simulink model "omx_joint_state_monitor"  (R2026a)
settings: Solver=VariableStepAuto  StopTime=Inf
libraries: ros2lib x2
settings Model: Creator=parkjuwon  LastModifiedBy=parkjuwon

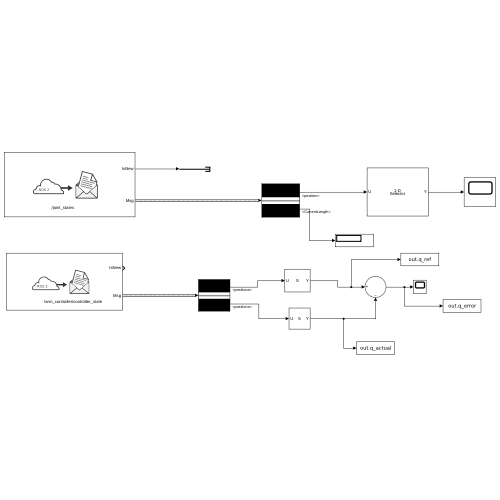
[thumbnail: Simulink's stored preview of the top-level diagram]
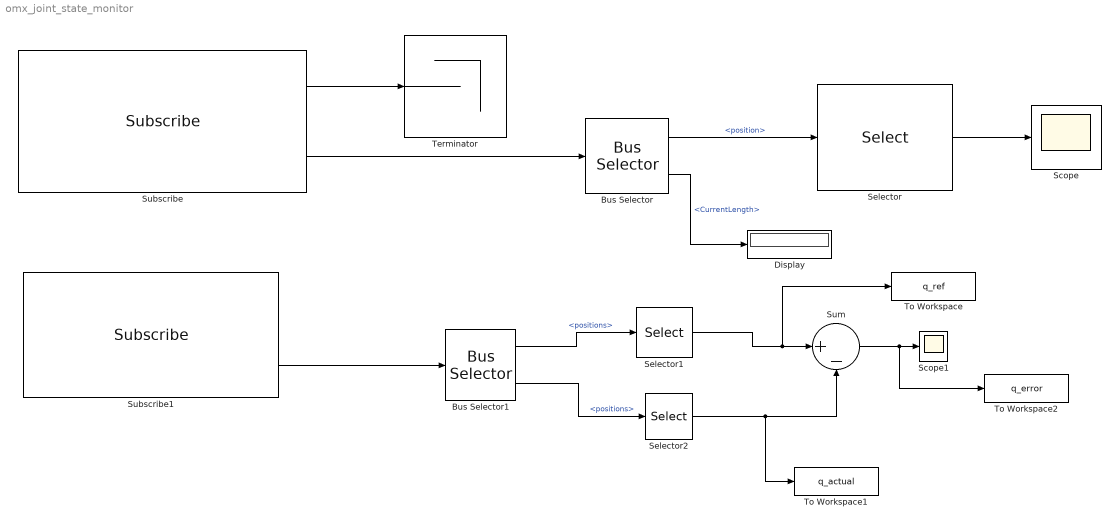
== system omx_joint_state_monitor ==
  Bus Selector : BusSelector  OutputSignals=position,position_SL_Info.CurrentLength
  Bus Selector1 : BusSelector  OutputSignals=reference.positions,feedback.positions
  Display : Display
  Scope : Scope
      settings: ActiveDisplayYMinimum=-1.1821267591514704  ActiveDisplayYMaximum=3.6890485001597582
  Scope1 : Scope
      settings: ActiveDisplayYMinimum=-6.9128041129529514  ActiveDisplayYMaximum=10.384679260876181
  Selector : Selector  IndexOptions=Index vector (dialog)  Indices=[3 4 5 6 7]  OutputSizes=1
  Selector1 : Selector  IndexOptions=Index vector (dialog)  Indices=[1 2 3 4 5]  OutputSizes=1
  Selector2 : Selector  IndexOptions=Index vector (dialog)  Indices=[1 2 3 4 5]  OutputSizes=1
  Subscribe : ros2lib/Subscribe  topicSource=Specify your own  topic=/joint_states  messageType=sensor_msgs/JointState  sampleTime=0.02  QOSHistory=Keep last  QOSDepth=10  QOSReliability=Reliable  QOSDurability=Volatile  QOSDeadline=Inf  QOSLifespan=Inf  QOSLiveliness=Automatic  QOSLeaseDuration=Inf  QOSAvoidROSNamespaceConventions=off
  Subscribe1 : ros2lib/Subscribe  topicSource=Specify your own  topic=/arm_controller/controller_state  messageType=control_msgs/JointTrajectoryControllerState  sampleTime=0.02  QOSHistory=Keep last  QOSDepth=10  QOSReliability=Reliable  QOSDurability=Volatile  QOSDeadline=Inf  QOSLifespan=Inf  QOSLiveliness=Automatic  QOSLeaseDuration=Inf  QOSAvoidROSNamespaceConventions=off
  Sum : Sum  Inputs=|+-
  Terminator : Terminator
  To Workspace : ToWorkspace  VariableName=q_ref  SaveFormat=Timeseries  SampleTime=-1
  To Workspace1 : ToWorkspace  VariableName=q_actual  SaveFormat=Timeseries  SampleTime=-1
  To Workspace2 : ToWorkspace  VariableName=q_error  SaveFormat=Timeseries  SampleTime=-1
  wires:
  Subscribe/2 -> Bus Selector/1
  Bus Selector/1 -> Selector/1  "<position>"
  Selector/1 -> Scope/1
  Subscribe/1 -> Terminator/1
  Bus Selector/2 -> Display/1  "<CurrentLength>"
  Bus Selector1/1 -> Selector1/1  "<positions>"
  Subscribe1/2 -> Bus Selector1/1
  Sum/1 -> To Workspace2/1, Scope1/1
  Bus Selector1/2 -> Selector2/1  "<positions>"
  Selector1/1 -> To Workspace/1, Sum/1
  Selector2/1 -> To Workspace1/1, Sum/2
